simulink model "PMSM_PI"  (R2024a)
settings: Solver=FixedStepAuto  StartTime=0.0  StopTime=10  FixedStep=TsModel  RelTol=1e-3
values from neighbouring files (symbols this model uses):
  ADRC_times = 4.0    [data_PMSM_PI.sldd]
  B = 0.0    [data_PMSM_PI.sldd]
  b0 = 2000.0    [data_PMSM_PI.sldd]
  CCR_Counter = 4199.0    [data_PMSM_PI.sldd]
  CUR_I = 105.0    [data_PMSM_PI.sldd]
  CUR_P = 0.255    [data_PMSM_PI.sldd]
  current_bandwidth = 1500.0    [data_PMSM_PI.sldd]
  currunt_omega_c = 350.0    [data_PMSM_PI.sldd]
  flux = 0.00419    [data_PMSM_PI.sldd]
  Idq_limit = 20.0    [data_PMSM_PI.sldd]
  J = 5.8E-5    [data_PMSM_PI.sldd]
  Ld = 0.00017    [data_PMSM_PI.sldd]
  Lq = 0.00017    [data_PMSM_PI.sldd]
  Ls = 0.00017    [data_PMSM_PI.sldd]
  omega_c = 330.0    [data_PMSM_PI.sldd]
  omega_c_LQR = 35.0    [data_PMSM_PI.sldd]
  PMSM_CCR_Counter = 4199.0    [data_PMSM_PI.sldd]
  Pn = 5.0    [data_PMSM_PI.sldd]
  Rs = 0.07    [data_PMSM_PI.sldd]
  speed_bandwidth = 200.0    [data_PMSM_PI.sldd]
  speed_bandwidth_LQR = 60.0    [data_PMSM_PI.sldd]
  SPEED_I = 18.457    [data_PMSM_PI.sldd]
  SPEED_P = 0.18457    [data_PMSM_PI.sldd]
  Ts = 0.0001    [data_PMSM_PI.sldd]
  TsModel = 2.5E-5    [data_PMSM_PI.sldd]
  two_b0 = 2649534.0    [data_PMSM_PI.sldd]
  two_omega_c = 85.0    [data_PMSM_PI.sldd]
undefined symbols (not defined in the file or in its folder): DiscIntNeverNeededParam, sigbuilder_block
libraries: slpidlib x4, simulink x1, mcbplantlib x1, autolibpmsmexterior x1
(part 1 of 2)
settings Model: DataDictionary=data_PMSM_PI.sldd  Creator=DaLiu  LastModifiedBy=ZJH
settings OptimizationCC: DefaultParameterBehavior=Inlined  GainParamInheritBuiltInType=on  UseFloatMulNetSlope=on  UseSpecifiedMinMax=on  InlineInvariantSignals=on  EnhancedBackFolding=on  PassReuseOutputArgsAs=Individual arguments  ZeroExternalMemoryAtStartup=off  NoFixptDivByZeroProtection=on  EfficientFloat2IntCast=on  OptimizeBlockOrder=speed  DifferentSizesBufferReuse=on  OptimizationCustomize=off  EfficientTunableParamExpr=on
settings DebuggingCC: ParameterOverflowMsg=none  ParameterUnderflowMsg=error  ParameterPrecisionLossMsg=none  ParameterTunabilityLossMsg=error
settings HardwareCC: ProdBitPerPointer=32  ProdBitPerSizeT=32  ProdBitPerPtrDiffT=32  ProdLargestAtomicInteger=Long  ProdLargestAtomicFloat=Double  ProdWordSize=32  ProdHWDeviceType=ARM Compatible->ARM Cortex-M
settings SFSimCC: MATLABDynamicMemAlloc=off
settings RTWCC: Description=Embedded Coder  SystemTargetFile=ert.tlc  GenCodeOnly=on  TemplateMakefile=ert_default_tmf  RTWUseSimCustomCode=on  BuildConfiguration=Faster Runs  GPUComputeCapability=3.5
settings CodeAppCC: ForceParamTrailComments=on  GenerateComments=off  IgnoreCustomStorageClasses=off  OperatorAnnotations=on  SimulinkDataObjDesc=on  SFDataObjDesc=on  InsertBlockDesc=on
settings ERTTargetCC: TargetLangStandard=C99 (ISO)  CodeReplacementLibrary=GNU C99 extensions  GenerateSampleERTMain=on  CombineSignalStateStructs=on  SupportAbsoluteTime=off  SupportNonFinite=off  SupportComplex=off  InlinedParameterPlacement=NonHierarchical  ERTCustomFileTemplate=example_file_process.tlc  IndentSize=4

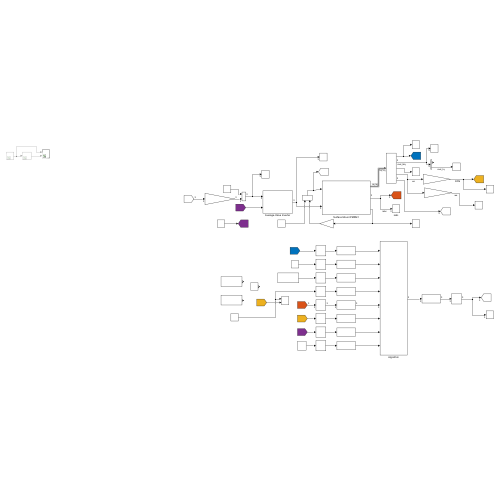
[thumbnail: Simulink's stored preview of the top-level diagram]
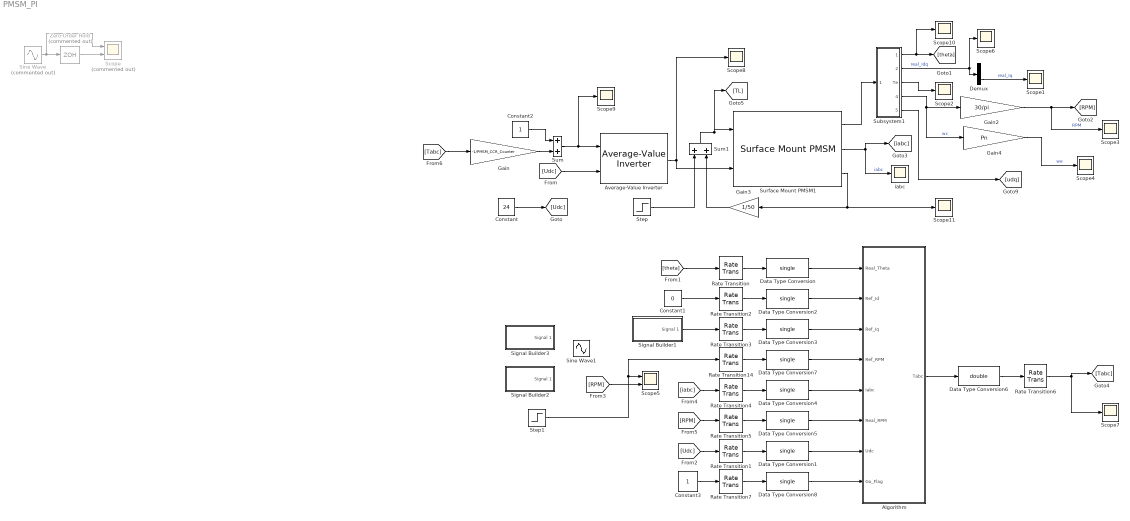
== system PMSM_PI ==
  Algorithm : Subsystem
  Average-Value Inverter : mcbplantlib/Average-Value Inverter
      settings: LibrarySourceBlock=mcblib/Electrical Systems/Inverters/Average-Value Inverter
  Constant : Constant  Value=24  SampleTime=TsModel
  Constant1 : Constant  Value=0  SampleTime=Ts
  Constant2 : Constant  SampleTime=TsModel
  Constant3 : Constant  SampleTime=Ts
  Data Type Conversion{,1..5,7..8} (8 alike) : DataTypeConversion  OutDataTypeStr=single  SaturateOnIntegerOverflow=off  RndMeth=Floor
  Data Type Conversion6 : DataTypeConversion  OutDataTypeStr=double  SaturateOnIntegerOverflow=off  RndMeth=Floor
  Demux : Demux  Outputs=2
  Gain : Gain  Gain=-1/PMSM_CCR_Counter
  Gain2 : Gain  Gain=30/pi
  Gain3 : Gain  Gain=1/50
  Gain4 : Gain  Gain=Pn
  Rate Transition{,1..5,7,14} (8 alike) : RateTransition  OutPortSampleTime=Ts
  Rate Transition6 : RateTransition  OutPortSampleTime=TsModel
  Scope : Scope  Commented=on  NumInputPorts=2
  Scope{1..4,6..11} (10 alike) : Scope
  Scope5 : Scope  NumInputPorts=2
  Signal Builder1 : Subsystem  Tag=STV Subsys  LoadFcn=sigbuilder_block('load');  StartFcn=sigbuilder_block('start');  StopFcn=sigbuilder_block('stop');  ClipboardFcn=sigbuilder_block('clipboard');  mask(Sigbuilder block){tuvar=[0:10]}
      mask help: Simulink:masks:SigbuilderBlock_MD
      mask init:
      | if ~strcmp(get_param(bdroot(gcbh),'SimulationStatus'),'stopped') tuvar = sigbuilder_block('maskInit'); end
      settings: CopyFcn=sigbuilder_block('copy');  DeleteFcn=sigbuilder_block('delete');  ModelCloseFcn=sigbuilder_block('modelClose');  PreSaveFcn=sigbuilder_block('preSave');  PauseFcn=sigbuilder_block('pause');  ContinueFcn=sigbuilder_block('continue');  NameChangeFcn=sigbuilder_block('namechange');  OpenFcn=sigbuilder_block('open',[192.6 154.8 702 251.4 ]);  CloseFcn=sigbuilder_block('close');
      mask Display: plot(0, 0, 100, 100,[2, 2, 32, 32, 2], [68, 8, 8, 68, 68],[32, 2], [38, 38], [32, 19, 2],[53, 60, 44], [32, 17, 17, 2],[16, 16, 31, 31]);txt = getActiveGroup(gcbh);text(2, 100, txt,'verticalAlignment', 'top');
  Signal Builder2 : Subsystem  Tag=STV Subsys  LoadFcn=sigbuilder_block('load');  StartFcn=sigbuilder_block('start');  StopFcn=sigbuilder_block('stop');  ClipboardFcn=sigbuilder_block('clipboard');  mask(Sigbuilder block){tuvar=[0:10]}
      mask help: Simulink:masks:SigbuilderBlock_MD
      mask init:
      | if ~strcmp(get_param(bdroot(gcbh),'SimulationStatus'),'stopped') tuvar = sigbuilder_block('maskInit'); end
      settings: CopyFcn=sigbuilder_block('copy');  DeleteFcn=sigbuilder_block('delete');  ModelCloseFcn=sigbuilder_block('modelClose');  PreSaveFcn=sigbuilder_block('preSave');  PauseFcn=sigbuilder_block('pause');  ContinueFcn=sigbuilder_block('continue');  NameChangeFcn=sigbuilder_block('namechange');  OpenFcn=sigbuilder_block('open',[205.2 81 729 231 ]);  CloseFcn=sigbuilder_block('close');
      mask Display: plot(0, 0, 100, 100,[2, 2, 32, 32, 2], [68, 8, 8, 68, 68],[32, 2], [38, 38], [32, 19, 2],[53, 60, 44], [32, 17, 17, 2],[16, 16, 31, 31]);txt = getActiveGroup(gcbh);text(2, 100, txt,'verticalAlignment', 'top');
  Signal Builder3 : Subsystem  Tag=STV Subsys  LoadFcn=sigbuilder_block('load');  StartFcn=sigbuilder_block('start');  StopFcn=sigbuilder_block('stop');  ClipboardFcn=sigbuilder_block('clipboard');  mask(Sigbuilder block){tuvar=[0:10]}
      mask help: Simulink:masks:SigbuilderBlock_MD
      mask init:
      | if ~strcmp(get_param(bdroot(gcbh),'SimulationStatus'),'stopped') tuvar = sigbuilder_block('maskInit'); end
      settings: CopyFcn=sigbuilder_block('copy');  DeleteFcn=sigbuilder_block('delete');  ModelCloseFcn=sigbuilder_block('modelClose');  PreSaveFcn=sigbuilder_block('preSave');  PauseFcn=sigbuilder_block('pause');  ContinueFcn=sigbuilder_block('continue');  NameChangeFcn=sigbuilder_block('namechange');  OpenFcn=sigbuilder_block('open',[303 127.2 729 342.6 ]);  CloseFcn=sigbuilder_block('close');
      mask Display: plot(0, 0, 100, 100,[2, 2, 32, 32, 2], [68, 8, 8, 68, 68],[32, 2], [38, 38], [32, 19, 2],[53, 60, 44], [32, 17, 17, 2],[16, 16, 31, 31]);txt = getActiveGroup(gcbh);text(2, 100, txt,'verticalAlignment', 'top');
  Sine Wave : Sin  Commented=on  SampleTime=Ts
  Sine Wave1 : Sin  Amplitude=150  SampleTime=0
  Step : Step  Time=5  After=0.1  SampleTime=Ts
  Step1 : Step  Time=0  After=100  SampleTime=Ts
  Subsystem1 : Subsystem
  Sum : Sum
  Sum1 : Sum
  Surface Mount PMSM1 : autolibpmsmexterior/Surface Mount PMSM  port_config=Torque  sim_type=Discrete  Ts=TsModel  P=Pn  Rs=Rs  Ldq_=Ls  KConstText=Permanent flux linkage constant (lambda_pm):  lambda_pm=flux  Ke=159.9771  Kt=1.323  mechanical=[J, B, 0]  idq0=[0 0]  theta_init=0  omega_init=0  KConst=flux  lambda_pm_calc=flux  RefBlkName='autolibpmsmexterior/Surface Mount PMSM'  aMode=5  Ldq="[0.0017      0.0017]"
  Zero-Order Hold : ZeroOrderHold  Commented=on
  iabc : Scope
  wires:
  Surface Mount PMSM1/1 -> Subsystem1/1(Info)
  Surface Mount PMSM1/2 -> [iabc], iabc/1  "iabc"
  Average-Value Inverter/1 -> Surface Mount PMSM1/2, Scope8/1
  Constant/1 -> [Udc]
  [Udc] -> Average-Value Inverter/2
  Subsystem1/2(I_dq) -> Demux/1, Scope6/1  "real_Idq"
  Demux/2 -> Scope1/1  "real_Iq"
  Subsystem1/3(Te) -> Scope2/1
  Subsystem1/4(Speed) -> Gain4/1, Gain2/1  "wc"
  Gain2/1 -> [RPM], Scope3/1  "RPM"
  Gain4/1 -> Scope4/1  "we"
  Subsystem1/1(Theta) -> [theta], Scope10/1
  [theta] -> Rate Transition/1
  Rate Transition/1 -> Data Type Conversion/1
  Data Type Conversion/1 -> Algorithm/1(Real_Theta)
  Data Type Conversion1/1 -> Algorithm/7(Udc)
  Rate Transition1/1 -> Data Type Conversion1/1
  [Udc] -> Rate Transition1/1
  Constant1/1 -> Rate Transition2/1
  Rate Transition2/1 -> Data Type Conversion2/1
  Data Type Conversion2/1 -> Algorithm/2(Ref_Id)
  Signal Builder1/1(Signal 1) -> Rate Transition3/1
  Data Type Conversion3/1 -> Algorithm/3(Ref_Iq)
  Rate Transition3/1 -> Data Type Conversion3/1
  Data Type Conversion7/1 -> Algorithm/4(Ref_RPM)
  Step1/1 -> Rate Transition14/1, Scope5/1
  [RPM] -> Scope5/2
  Rate Transition14/1 -> Data Type Conversion7/1
  [iabc] -> Rate Transition4/1
  Rate Transition4/1 -> Data Type Conversion4/1
  Data Type Conversion4/1 -> Algorithm/5(Iabc)
  [RPM] -> Rate Transition5/1
  Rate Transition5/1 -> Data Type Conversion5/1
  Data Type Conversion5/1 -> Algorithm/6(Real_RPM)
  Algorithm/1(Tabc) -> Data Type Conversion6/1
  Data Type Conversion6/1 -> Rate Transition6/1
  Rate Transition6/1 -> [Tabc], Scope7/1
  [Tabc] -> Gain/1
  Gain/1 -> Sum/2
  Constant2/1 -> Sum/1
  Sum/1 -> Scope9/1, Average-Value Inverter/1
  Surface Mount PMSM1/3 -> Scope11/1, Gain3/1
  Constant3/1 -> Rate Transition7/1
  Rate Transition7/1 -> Data Type Conversion8/1
  Data Type Conversion8/1 -> Algorithm/8(Go_Flag)
  Step/1 -> Sum1/1
  Gain3/1 -> Sum1/2
  Sum1/1 -> [TL], Surface Mount PMSM1/1
  Subsystem1/5(udq) -> [udq]
  Sine Wave/1 -> Scope/1, Zero-Order Hold/1
  Zero-Order Hold/1 -> Scope/2

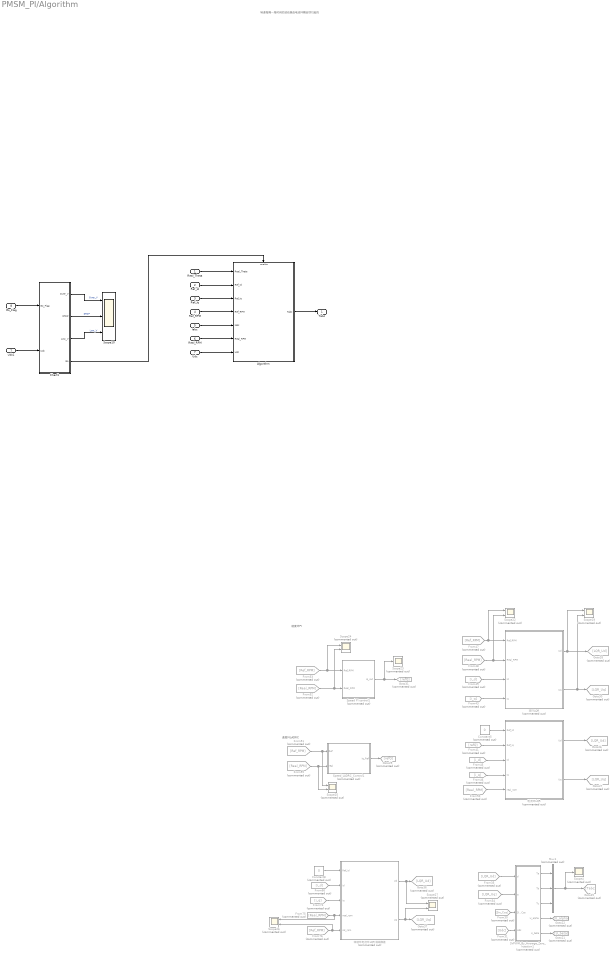
== system PMSM_PI/Algorithm ==
  note: 转速每隔一段时间的波动是由电流环耦合项引起的
  note: 速度环LADRC
  note: 速度环PI
  Real_Theta : Inport  OutDataTypeStr=single
  Ref_Id : Inport  Port=2  OutDataTypeStr=single
  Ref_Iq : Inport  Port=3  OutDataTypeStr=single
  Ref_RPM : Inport  Port=4  OutDataTypeStr=single
  Iabc : Inport  Port=5  OutDataTypeStr=single
  Real_RPM : Inport  Port=6
  Udc : Inport  Port=7  OutDataTypeStr=single
  Go_Flag : Inport  Port=8
  Algorithm : Subsystem
  Chart1 : Stateflow chart  TreatAsAtomicUnit=on
  Constant5 : Constant  Commented=on  Value=0  SampleTime=Ts
  Constant8 : Constant  Commented=on  Value=0  SampleTime=Ts
  From30 : From  Commented=on  GotoTag=Sin_Cos
  From31 : From  Commented=on  GotoTag=Udc
  From34 : From  Commented=on  GotoTag=LQR_Uq
  From35 : From  Commented=on  GotoTag=LQR_Ud
  From41 : From  Commented=on  GotoTag=refQ
  From43 : From  Commented=on  GotoTag=i_q
  From45 : From  Commented=on  GotoTag=i_d
  From46 : From  Commented=on  GotoTag=i_q
  From{47,51,53,76} (4 alike) : From  Commented=on  GotoTag=Ref_RPM
  From{48,50,52,55,75} (5 alike) : From  Commented=on  GotoTag=Real_RPM
  From49 : From  Commented=on  GotoTag=i_d
  From66 : From  Commented=on  GotoTag=i_d
  From74 : From  Commented=on  GotoTag=i_q
  Goto21 : Goto  Commented=on  GotoTag=U_beta
  Goto22 : Goto  Commented=on  GotoTag=U_alpha
  Goto25 : Goto  Commented=on  GotoTag=Tabc
  Goto26 : Goto  Commented=on  GotoTag=LQR_Ud
  Goto27 : Goto  Commented=on  GotoTag=LQR_Uq
  Goto28 : Goto  Commented=on  GotoTag=LQR_Ud
  Goto29 : Goto  Commented=on  GotoTag=refQ
  Goto30 : Goto  Commented=on  GotoTag=LQR_Uq
  Goto31 : Goto  Commented=on  GotoTag=refQ
  Goto36 : Goto  Commented=on  GotoTag=LQR_Ud
  Goto37 : Goto  Commented=on  GotoTag=LQR_Uq
  Mux1 : Mux  Commented=on  Inputs=3
  SVPWM_By_Average_Zero_Injection1 : Subsystem  Commented=on  TreatAsAtomicUnit=on
  Scope10 : Scope  NumInputPorts=3
  Scope{19,22,24..27} (6 alike) : Scope  Commented=on  NumInputPorts=2
  Scope23 : Scope  Commented=on
  Scope4 : Scope  Commented=on
  Speed PI control1 : Subsystem  Commented=on  TreatAsAtomicUnit=on
  Speed_LADRC_Control1 : Subsystem  Commented=on  TreatAsAtomicUnit=on
  Udc1 : InportShadow  Port=7  OutDataTypeStr=single
  双环LQR : Subsystem  Commented=on
  电流环LQR : Subsystem  Commented=on
  转速环电流环LQR消除静差 : Subsystem  Commented=on
  Tabc : Outport  OutDataTypeStr=single
  wires:
  Udc/1 -> Algorithm/7(Udc)
  Real_Theta/1 -> Algorithm/1(Real_Theta)
  Ref_RPM/1 -> Algorithm/4(Ref_RPM)
  Ref_Iq/1 -> Algorithm/3(Ref_Iq)
  Iabc/1 -> Algorithm/5(Iabc)
  Real_RPM/1 -> Algorithm/6(Real_RPM)
  Mux1/1 -> Goto25/1, Scope4/1
  SVPWM_By_Average_Zero_Injection1/3(Tc) -> Mux1/3
  SVPWM_By_Average_Zero_Injection1/5(U_beta) -> Goto21/1
  SVPWM_By_Average_Zero_Injection1/2(Tb) -> Mux1/2
  SVPWM_By_Average_Zero_Injection1/4(U_alpha) -> Goto22/1
  SVPWM_By_Average_Zero_Injection1/1(Ta) -> Mux1/1
  From35/1 -> SVPWM_By_Average_Zero_Injection1/1(d)
  From30/1 -> SVPWM_By_Average_Zero_Injection1/3(Sin&Cos)
  From31/1 -> SVPWM_By_Average_Zero_Injection1/4(Udc)
  From34/1 -> SVPWM_By_Average_Zero_Injection1/2(q)
  Algorithm/1(Tabc) -> Tabc/1
  From48/1 -> Scope22/2, 双环LQR/2(Real_RPM)
  From47/1 -> Scope22/1, 双环LQR/1(Ref_RPM)
  From49/1 -> 双环LQR/3(id)
  From43/1 -> 双环LQR/4(iq)
  双环LQR/2(Uq) -> Scope19/2, Goto30/1
  双环LQR/1(Ud) -> Scope19/1, Goto28/1
  电流环LQR/1(Ud) -> Goto26/1
  电流环LQR/2(Uq) -> Goto27/1
  From41/1 -> 电流环LQR/2(Ref_iq)
  Constant5/1 -> 电流环LQR/1(Ref_id)
  From45/1 -> 电流环LQR/3(id)
  From46/1 -> 电流环LQR/4(iq)
  From50/1 -> 电流环LQR/5(real_rpm)
  From52/1 -> Speed PI control1/2(Real_RPM), Scope24/2
  From53/1 -> Speed PI control1/1(Ref_RPM), Scope24/1
  From51/1 -> Speed_LADRC_Control1/1(Ref), Scope25/1
  Speed PI control1/1(Iq_out) -> Goto31/1, Scope23/1
  From55/1 -> Scope25/2, Speed_LADRC_Control1/2(real)
  Speed_LADRC_Control1/1(Iq_Ref) -> Goto29/1
  From76/1 -> Scope26/2, 转速环电流环LQR消除静差/5(rel_rpm)
  From75/1 -> Scope26/1, 转速环电流环LQR消除静差/4(real_rpm)
  From74/1 -> 转速环电流环LQR消除静差/3(iq)
  From66/1 -> 转速环电流环LQR消除静差/2(id)
  Constant8/1 -> 转速环电流环LQR消除静差/1(Ref_id)
  转速环电流环LQR消除静差/2(Uq) -> Scope27/2, Goto37/1
  转速环电流环LQR消除静差/1(Ud) -> Scope27/1, Goto36/1
  Go_Flag/1 -> Chart1/1(Go_Flag)
  Chart1/3(Low_V) -> Scope10/3  "Low_V"
  Chart1/2(STOP) -> Scope10/2  "STOP"
  Chart1/1(Over_V) -> Scope10/1  "Over_V"
  Udc1/1 -> Chart1/2(Udc)
  Chart1/4(Go) -> Algorithm/Enable
  Ref_Id/1 -> Algorithm/2(Ref_Id)

== system PMSM_PI/Signal Builder1 ==
  Demux : Demux  Tag=STV Demux  Outputs=1
      settings: DisplayOption=none
  FromWs : FromWorkspace  Tag=STV FromWs  VariableName=tuvar
      SigBuilderData=|
      | common.afterFinalStr = 'Extrapolate'
      | common.sampleTime = 0
      | dataSet.timeRange = [0 10]
      | dataSet.name = 'Group 1'
      | sbobj.Groups.Name = 'Group 1'
      | sbobj.Groups.Signals.Name = 'Signal 1'
      | sbobj.Groups.Signals.XData = [0 1.9 1.9 3.56 3.56 10]
      | sbobj.Groups.Signals.YData = [5 5 7.2 7.2 8 8]
  Signal 1 : Outport  Tag=STV Outport
  wires:
  Demux/1 -> Signal 1/1
  FromWs/1 -> Demux/1

== system PMSM_PI/Signal Builder2 ==
  Demux : Demux  Tag=STV Demux  Outputs=1
      settings: DisplayOption=none
  FromWs : FromWorkspace  Tag=STV FromWs  VariableName=tuvar
      SigBuilderData=|
      | common.afterFinalStr = 'Extrapolate'
      | common.sampleTime = 0
      | dataSet.timeRange = [0 10]
      | dataSet.name = 'Group 1'
      | sbobj.Groups.Name = 'Group 1'
      | sbobj.Groups.Signals.Name = 'Signal 1'
      | sbobj.Groups.Signals.XData = [0 3 6.02 10]
      | sbobj.Groups.Signals.YData = [150 150 250 200]
  Signal 1 : Outport  Tag=STV Outport
  wires:
  Demux/1 -> Signal 1/1
  FromWs/1 -> Demux/1

== system PMSM_PI/Signal Builder3 ==
  Demux : Demux  Tag=STV Demux  Outputs=1
      settings: DisplayOption=none
  FromWs : FromWorkspace  Tag=STV FromWs  VariableName=tuvar
      SigBuilderData=|
      | common.afterFinalStr = 'Extrapolate'
      | common.sampleTime = 0
      | dataSet.timeRange = [0 10]
      | dataSet.name = 'Group 1'
      | sbobj.Groups.Name = 'Group 1'
      | sbobj.Groups.Signals.Name = 'Signal 1'
      | sbobj.Groups.Signals.XData = [0 3 3 6.02 6.02 10]
      | sbobj.Groups.Signals.YData = [150 150 250 250 200 200]
  Signal 1 : Outport  Tag=STV Outport
  wires:
  FromWs/1 -> Demux/1
  Demux/1 -> Signal 1/1

== system PMSM_PI/Subsystem1 ==
  Info : Inport
  Bus Selector2 : BusSelector  OutputSignals=IdSync,IqSync,MtrPos,MtrTrq,MtrSpd,VdSync,VqSync
  Constant4 : Constant  Value=2*pi  SampleTime=-1
  Gain2 : Gain  Gain=Pn
  Mod1 : Math  Operator=mod
  Mux : Mux  Inputs=2
  Mux1 : Mux  Inputs=2
  Scope : Scope
  Theta : Outport
  I_dq : Outport  Port=2
  Te : Outport  Port=3
  Speed : Outport  Port=4
  udq : Outport  Port=5
  wires:
  Bus Selector2/2 -> Mux/2  "<IqSync>"
  Gain2/1 -> Mod1/1
  Mod1/1 -> Theta/1
  Bus Selector2/1 -> Mux/1  "<IdSync>"
  Constant4/1 -> Mod1/2
  Info/1 -> Bus Selector2/1
  Bus Selector2/3 -> Gain2/1  "<MtrPos>"
  Mux/1 -> I_dq/1
  Bus Selector2/4 -> Te/1  "<MtrTrq>"
  Bus Selector2/5 -> Scope/1, Speed/1  "<MtrSpd>"
  Bus Selector2/6 -> Mux1/1  "<VdSync>"
  Bus Selector2/7 -> Mux1/2  "<VqSync>"
  Mux1/1 -> udq/1

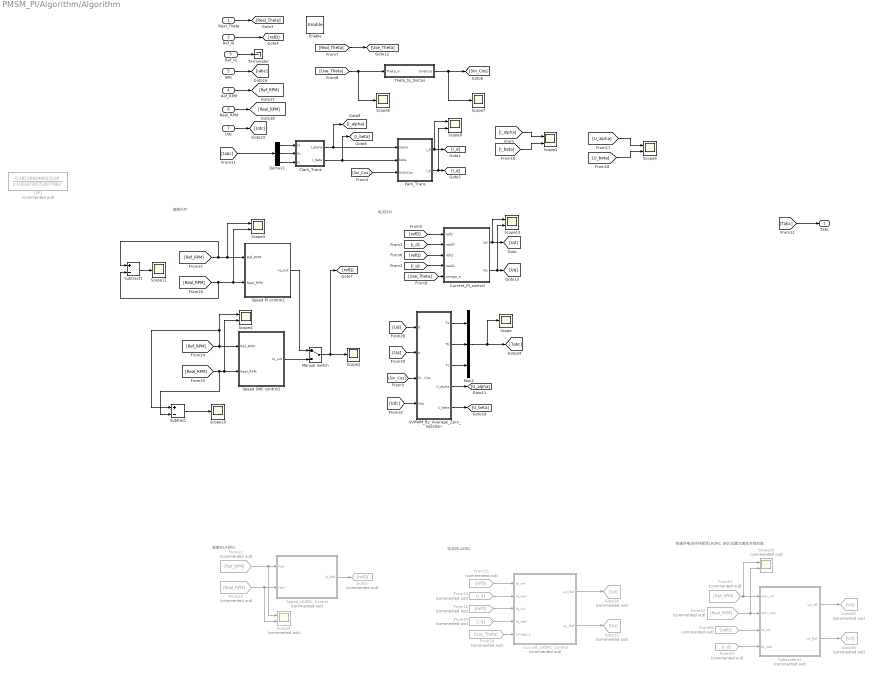
== system PMSM_PI/Algorithm/Algorithm ==
  note: 电流环PI
  note: 速度环PI
  note: 转速环电流环并联双LADRC
      | 该b0设置为真实方程的值
  note: 电流环LADRC
  note: 速度环LADRC
  Real_Theta : Inport  OutDataTypeStr=single
  Ref_Id : Inport  Port=2  OutDataTypeStr=single
  Ref_Iq : Inport  Port=3  OutDataTypeStr=single
  Ref_RPM : Inport  Port=4  OutDataTypeStr=single
  Iabc : Inport  Port=5  OutDataTypeStr=single
  Real_RPM : Inport  Port=6
  Udc : Inport  Port=7  OutDataTypeStr=single
  Enable : EnablePort
  Clark_Trans : Subsystem  TreatAsAtomicUnit=on
      settings: RTWFcnNameOpts=Use subsystem name
  Current_PI_control : Subsystem  TreatAsAtomicUnit=on
      settings: RTWFcnNameOpts=Use subsystem name
  Currunt_LADRC_Control : Subsystem  Commented=on
  Demux1 : Demux  Outputs=3
  From13 : From  Commented=on  GotoTag=i_d
  From14 : From  Commented=on  GotoTag=i_q
  From15 : From  Commented=on  GotoTag=refD
  From16 : From  Commented=on  GotoTag=refQ
  From19 : From  Commented=on  GotoTag=Use_Theta
  From22 : From  Commented=on  GotoTag=Ref_RPM
  From23 : From  Commented=on  GotoTag=Real_RPM
  From37 : From  Commented=on  GotoTag=Real_RPM
  From54 : From  Commented=on  GotoTag=Ref_RPM
  From56 : From  Commented=on  GotoTag=refD
  From57 : From  Commented=on  GotoTag=i_d
  Goto14 : Goto  Commented=on  GotoTag=Ud
  Goto15 : Goto  Commented=on  GotoTag=Uq
  Goto38 : Goto  Commented=on  GotoTag=Ud
  Goto39 : Goto  Commented=on  GotoTag=Uq
  Goto5 : Goto  Commented=on  GotoTag=refQ
  LPF1 : DiscreteTransferFcn  Commented=on  Numerator=[0.181269246922018]  Denominator=[1 -0.818730753077982]
  Manual Switch : ManualSwitch
  Mux2 : Mux  Inputs=3
  Park_Trans : Subsystem  TreatAsAtomicUnit=on
      settings: RTWFcnNameOpts=Use subsystem name
  SVPWM_By_Average_Zero_Injection : Subsystem  TreatAsAtomicUnit=on
  Scope{,2,6..7,10..11} (6 alike) : Scope
  Scope{1,3..4,8..9,13} (6 alike) : Scope  NumInputPorts=2
  Scope29 : Scope  Commented=on  NumInputPorts=2
  Scope5 : Scope  Commented=on  NumInputPorts=2
  Speed PI control2 : Subsystem  TreatAsAtomicUnit=on
  Speed SMC control1 : Subsystem  TreatAsAtomicUnit=on
  Speed_LADRC_Control : Subsystem  Commented=on  TreatAsAtomicUnit=on
  Subsystem1 : Subsystem  Commented=on
  Subtract : Sum  Inputs=+-
  Subtract1 : Sum  Inputs=+-
  Terminator : Terminator
  Theta_to_SinCos : Subsystem  TreatAsAtomicUnit=on
  Tabc : Outport
  wires:
  [i_d] -> Current_PI_control/2(realD)
  [refQ] -> Current_PI_control/3(refQ)
  [Udc] -> SVPWM_By_Average_Zero_Injection/4(Udc)
  SVPWM_By_Average_Zero_Injection/3(Tc) -> Mux2/3
  Current_PI_control/1(Ud) -> Scope13/1, [Ud]
  [Uq] -> SVPWM_By_Average_Zero_Injection/2(q)
  [refD] -> Current_PI_control/1(refD)
  [Sin_Cos] -> SVPWM_By_Average_Zero_Injection/3(Sin&Cos)
  Mux2/1 -> [Tabc], Scope/1
  SVPWM_By_Average_Zero_Injection/4(U_alpha) -> [U_alpha]
  Current_PI_control/2(Uq) -> Scope13/2, [Uq]
  [Ud] -> SVPWM_By_Average_Zero_Injection/1(d)
  [Ref_RPM] -> Subtract1/1, Scope3/1, Speed PI control2/1(Ref_RPM)
  SVPWM_By_Average_Zero_Injection/1(Ta) -> Mux2/1
  [i_q] -> Current_PI_control/4(realQ)
  [Real_RPM] -> Speed PI control2/2(Real_RPM), Scope3/2, Subtract1/2
  SVPWM_By_Average_Zero_Injection/5(U_beta) -> [U_beta]
  SVPWM_By_Average_Zero_Injection/2(Tb) -> Mux2/2
  [Use_Theta] -> Current_PI_control/5(omega_e)
  [Sin_Cos] -> Park_Trans/3(Sin&Cos)
  Clark_Trans/1(I_alpha) -> [I_alpha], Park_Trans/1(alpha)
  [I_alpha] -> Scope1/1
  Park_Trans/1(i_d) -> Scope8/1, [i_d]
  Clark_Trans/2(I_beta) -> Park_Trans/2(beta), [I_beta]
  Demux1/1 -> Clark_Trans/1(Ia)
  [Use_Theta] -> Scope6/1, Theta_to_SinCos/1(Theta_in)
  [Real_Theta] -> [Use_Theta]
  Theta_to_SinCos/1(Sin&Cos) -> Scope7/1, [Sin_Cos]
  [U_alpha] -> Scope9/1
  Park_Trans/2(i_q) -> Scope8/2, [i_q]
  Demux1/3 -> Clark_Trans/3(Ic)
  [U_beta] -> Scope9/2
  Demux1/2 -> Clark_Trans/2(Ib)
  [I_beta] -> Scope1/2
  Ref_Id/1 -> [refD]
  Real_Theta/1 -> [Real_Theta]
  Ref_Iq/1 -> Terminator/1
  Iabc/1 -> [Iabc]
  Real_RPM/1 -> [Real_RPM]
  Ref_RPM/1 -> [Ref_RPM]
  Udc/1 -> [Udc]
  [Tabc] -> Tabc/1
  From16/1 -> Currunt_LADRC_Control/3(Iq_ref)
  From14/1 -> Currunt_LADRC_Control/4(Iq_real)
  Speed_LADRC_Control/1(Iq_Ref) -> Goto5/1
  From54/1 -> Scope29/1, Subsystem1/1(rpm_ref)
  Subsystem1/1(uq_ref) -> Goto39/1
  From23/1 -> Speed_LADRC_Control/2(real), Scope5/2
  From57/1 -> Subsystem1/4(Id_real)
  From37/1 -> Scope29/2, Subsystem1/2(rpm_real)
  From13/1 -> Currunt_LADRC_Control/2(Id_real)
  From22/1 -> Scope5/1, Speed_LADRC_Control/1(Ref)
  From19/1 -> Currunt_LADRC_Control/5(omega_e)
  Subsystem1/2(ud_Ref) -> Goto38/1
  Currunt_LADRC_Control/2(uq_Ref) -> Goto15/1
  From15/1 -> Currunt_LADRC_Control/1(Id_ref)
  Currunt_LADRC_Control/1(ud_Ref) -> Goto14/1
  From56/1 -> Subsystem1/3(Id_ref)
  [Iabc] -> Demux1/1
  Speed PI control2/1(Iq_out) -> Manual Switch/1
  Manual Switch/1 -> [refQ], Scope2/1
  Speed SMC control1/1(Iq_out) -> Manual Switch/2
  [Real_RPM] -> Subtract/2, Scope4/2, Speed SMC control1/2(Real_RPM)
  [Ref_RPM] -> Scope4/1, Subtract/1, Speed SMC control1/1(Ref_RPM)
  Subtract/1 -> Scope10/1
  Subtract1/1 -> Scope11/1

== system PMSM_PI/Algorithm/Chart1/Low_judge ==
  Input : Inport  OutDataTypeStr=single  PortDimensions=1
  f : TriggerPort  TriggerType=function-call  VariantControl=(inherit)
      settings: CopyFcn=Stateflow.SLINSF.SimulinkMan.removeBlockPreDeleteFcn  PreDeleteFcn=Stateflow.SLINSF.SimulinkMan.unsafePredeleteFcn
  Data Type Conversion : DataTypeConversion  OutDataTypeStr=boolean  SaturateOnIntegerOverflow=off  RndMeth=Floor
  Data Type Conversion1 : DataTypeConversion  OutDataTypeStr=single  SaturateOnIntegerOverflow=off  RndMeth=Floor
  NOR : Logic  Operator=NOT  IconShape=distinctive  OutDataTypeStr=boolean
  Relay : Relay  OnSwitchValue=20  OffSwitchValue=18  OutDataTypeStr=single
  Out : Outport  OutDataTypeStr=single
  wires:
  Input/1 -> Relay/1
  Relay/1 -> Data Type Conversion/1
  NOR/1 -> Data Type Conversion1/1
  Data Type Conversion/1 -> NOR/1
  Data Type Conversion1/1 -> Out/1

== system PMSM_PI/Algorithm/Chart1/Over_judge ==
  Input : Inport  OutDataTypeStr=single  PortDimensions=1
  f : TriggerPort  TriggerType=function-call  VariantControl=(inherit)
      settings: CopyFcn=Stateflow.SLINSF.SimulinkMan.removeBlockPreDeleteFcn  PreDeleteFcn=Stateflow.SLINSF.SimulinkMan.unsafePredeleteFcn
  Relay : Relay  OnSwitchValue=28  OffSwitchValue=25  OutDataTypeStr=single
  Out : Outport  OutDataTypeStr=single
  wires:
  Input/1 -> Relay/1
  Relay/1 -> Out/1

== system PMSM_PI/Algorithm/SVPWM_By_Average_Zero_Injection1 ==
  d : Inport  OutDataTypeStr=single
  q : Inport  Port=2  OutDataTypeStr=single
  Sin&Cos : Inport  Port=3  OutDataTypeStr=single
  Udc : Inport  Port=4  OutDataTypeStr=single
  Anti_Park_Trans : Subsystem
  Gain : Gain  Gain=CCR_Counter  OutDataTypeStr=single
  Gain1 : Gain  Gain=CCR_Counter  OutDataTypeStr=single
  Gain2 : Gain  Gain=CCR_Counter  OutDataTypeStr=single
  SVPWM : Subsystem
  Scope : Scope  NumInputPorts=3
  Ta : Outport  OutDataTypeStr=single
  Tb : Outport  Port=2  OutDataTypeStr=single
  Tc : Outport  Port=3  OutDataTypeStr=single
  U_alpha : Outport  Port=4  OutDataTypeStr=single
  U_beta : Outport  Port=5  OutDataTypeStr=single
  wires:
  Anti_Park_Trans/1(alpha) -> U_alpha/1, SVPWM/1(alpha)
  q/1 -> Anti_Park_Trans/2(q)
  SVPWM/1(Ta) -> Scope/1, Gain/1
  Anti_Park_Trans/2(beta) -> U_beta/1, SVPWM/2(beta)
  d/1 -> Anti_Park_Trans/1(d)
  Sin&Cos/1 -> Anti_Park_Trans/3(Sin&Cos)
  SVPWM/2(Tb) -> Scope/2, Gain1/1
  SVPWM/3(Tc) -> Gain2/1, Scope/3
  Udc/1 -> SVPWM/3(Udc)
  Gain/1 -> Ta/1
  Gain1/1 -> Tb/1
  Gain2/1 -> Tc/1

== system PMSM_PI/Algorithm/Speed PI control1 ==
  Ref_RPM : Inport  OutDataTypeStr=single
  Real_RPM : Inport  Port=2  OutDataTypeStr=single
  Add : Sum  Inputs=+-  OutDataTypeStr=single
  Constant1 : Constant  Value=speed_bandwidth_LQR  OutDataTypeStr=single  SampleTime=Ts
  Constant2 : Constant  Value=speed_bandwidth_LQR  OutDataTypeStr=single  SampleTime=Ts
  Constant3 : Constant  Value=B  OutDataTypeStr=single  SampleTime=Ts
  Constant4 : Constant  Value=1.5*Pn*flux  OutDataTypeStr=single  SampleTime=Ts
  Divide : Product  Inputs=*/  OutDataTypeStr=single
  Gain : Gain  Gain=J/(1.5*Pn*flux)  OutDataTypeStr=single
  Gain1 : Gain  Gain=J/(1.5*Pn*flux)  OutDataTypeStr=single
  Gain2 : Gain  Gain=J  OutDataTypeStr=single
  PID Controller : slpidlib/PID Controller  Controller=PI  Form=Parallel  TimeDomain=Discrete-time  UseExternalTs=off  SampleTime=Ts  IntegratorMethod=Forward Euler  FilterMethod=Forward Euler  ControllerParametersSource=external  P=1  I=1  UseKiTs=off  D=0  UseExternalDerivativeSource=off  N=100  UseFilter=on  TunerSelectOption=Transfer Function Based (PID Tuner App)  ZeroCross=off  InitialConditionSource=internal  InitialConditionForIntegrator=1  InitialConditionForFilter=0  DifferentiatorICPrevScaledInput=0  ExternalReset=none  TrackingMode=off  Kt=1  LimitOutput=off  SatLimitsSource=internal  UpperSaturationLimit=200  LowerSaturationLimit=-200  LinearizeAsGain=on  AntiWindupMode=none  Kb=1  LimitIntegrator=off  UpperIntegratorSaturationLimit=inf  LowerIntegratorSaturationLimit=-inf  POutMin=[]  POutMax=[]  IOutMin=[]  IOutMax=[]  DOutMin=[]  DOutMax=[]  NOutMin=[]  NOutMax=[]  SumOutMin=[]  SumOutMax=[]  SaturationOutMin=[]  SaturationOutMax=[]  PParamMin=[]  PParamMax=[]  IParamMin=[]  IParamMax=[]  DParamMin=[]  DParamMax=[]  NParamMin=[]  NParamMax=[]  KbParamMin=[]  KbParamMax=[]  KtParamMin=[]  KtParamMax=[]  KbOutMin=[]  KbOutMax=[]  KtOutMin=[]  KtOutMax=[]  IntegratorOutMin=[]  IntegratorOutMax=[]  FilterOutMin=[]  FilterOutMax=[]  SumI1OutMin=[]  SumI1OutMax=[]  SumI2OutMin=[]  SumI2OutMax=[]  SumI3OutMin=[]  SumI3OutMax=[]  SumI4OutMin=[]  SumI4OutMax=[]  SumDOutMin=[]  SumDOutMax=[]  DifferentiatorOutMin=[]  DifferentiatorOutMax=[]  FilterDiffOutCoefMin=[]  FilterDiffOutCoefMax=[]  ReciprocalOutMin=[]  ReciprocalOutMax=[]  SumDenOutMin=[]  SumDenOutMax=[]  SumNumOutMin=[]  SumNumOutMax=[]  DivideOutMin=[]  DivideOutMax=[]  UdiffTsProdOutMin=[]  UdiffTsProdOutMax=[]  NTsProdOutMin=[]  NTsProdOutMax=[]  UintegralTsProdOutMin=[]  UintegralTsProdOutMax=[]  UngainTsProdOutMin=[]  UngainTsProdOutMax=[]  ClampingZeroOutDataTypeStr=Inherit: Inherit via back propagation  ClampingZeroOutMin=[]  ClampingZeroOutMax=[]  FilterDenConstantOutDataTypeStr=Inherit: Inherit via back propagation  FilterDenConstantOutMin=[]  FilterDenConstantOutMax=[]  PCopyOutDataTypeStr=Inherit: Inherit via back propagation  PCopyOutMin=[]  PCopyOutMax=[]  NCopyOutDataTypeStr=Inherit: Inherit via back propagation  NCopyOutMin=[]  NCopyOutMax=[]  IntegratorContinuousStateAttributes=''  IntegratorStateMustResolveToSignalObject=off  IntegratorRTWStateStorageClass=Auto  FilterContinuousStateAttributes=''  FilterStateMustResolveToSignalObject=off  FilterRTWStateStorageClass=Auto  ParallelPVariant=ExternalParameters  IdealPVariant=Disabled  IVariant=ExternalParameters  DVariant=Disabled  IntegratorVariant=Discrete  SatVariant=Disabled  AWVariant=Passthrough  PCopyVariant=Disabled  TRVariant=Disabled  FdbkBlocksVariant=Forward  IdealPFdbkVariant=Disabled  SatFdbkVariant=Disabled  DerivativeFilterVariant=Disabled  NVariant=Disabled  NCopyVariant=Disabled_SignalSpec  FilterICVariant=Disabled  IntegratorICVariant=InternalICs  ExternalResetVariant=Disabled  TRSumVariant=Passthrough  SumFdbkVariant=Disabled  SumVariant=Sum_PI  TsampFilterVariant=InternalTs  TsampNgainVariant=Passthrough  TsampIntegralVariant=Disabled_SignalSpec  ExternalSaturationOutDataTypeStr=Inherit: Same as second input  DerivativeSourceVariant=Disabled
  Product : Product  OutDataTypeStr=single
  Product1 : Product  OutDataTypeStr=single
  Saturation2 : Saturate  UpperLimit=Idq_limit  LowerLimit=-Idq_limit  OutDataTypeStr=single
  Step : Step  Time=8  After=0  SampleTime=Ts
  Sum : Sum  Inputs=|++
  Sum1 : Sum  Inputs=|+-  OutDataTypeStr=single
  Sum2 : Sum  Inputs=|+-  OutDataTypeStr=single
  Iq_out : Outport  OutDataTypeStr=single
  wires:
  Step/1 -> Sum/2
  Sum/1 -> Saturation2/1
  Saturation2/1 -> Iq_out/1
  Sum2/1 -> Sum/1
  Product1/1 -> Sum2/2
  Divide/1 -> Product1/1
  Constant4/1 -> Divide/2
  Add/1 -> Divide/1
  Constant3/1 -> Add/2
  Gain2/1 -> Add/1
  Product/1 -> Gain1/1
  Gain1/1 -> PID Controller/3
  Constant2/1 -> Product/1, Product/2, Gain2/1
  PID Controller/1 -> Sum2/1
  Real_RPM/1 -> Product1/2, Sum1/2
  Sum1/1 -> PID Controller/1
  Ref_RPM/1 -> Sum1/1
  Gain/1 -> PID Controller/2
  Constant1/1 -> Gain/1

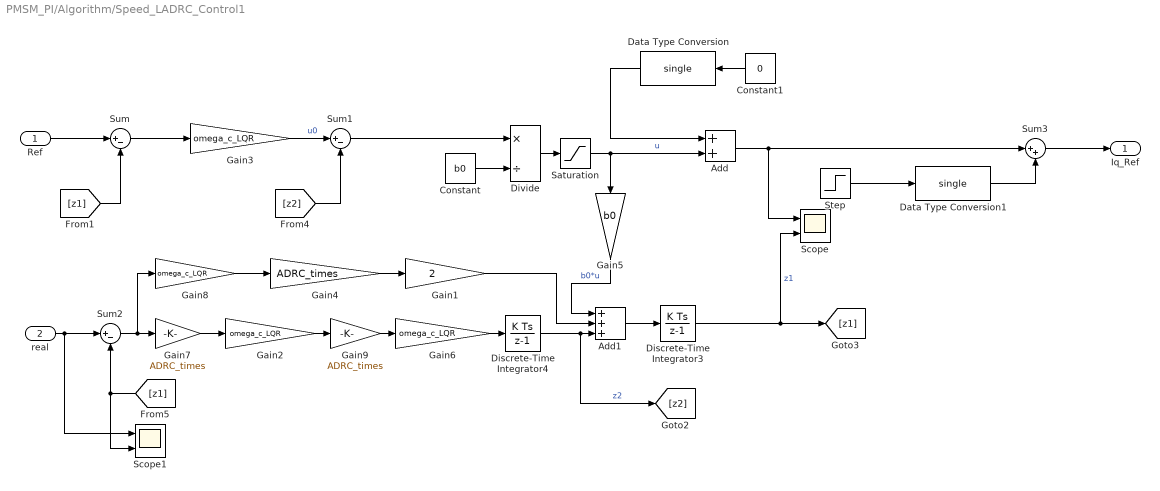
== system PMSM_PI/Algorithm/Speed_LADRC_Control1 ==
  Ref : Inport  OutDataTypeStr=single
  real : Inport  Port=2  OutDataTypeStr=single
  Add : Sum  OutDataTypeStr=single
  Add1 : Sum  Inputs=+++  OutDataTypeStr=single
  Constant : Constant  Value=b0  OutDataTypeStr=single
  Constant1 : Constant  Value=0  SampleTime=-1
  Data Type Conversion : DataTypeConversion  OutDataTypeStr=single  SaturateOnIntegerOverflow=off  RndMeth=Floor
  Data Type Conversion1 : DataTypeConversion  OutDataTypeStr=single  SaturateOnIntegerOverflow=off  RndMeth=Floor
  Discrete-Time Integrator3 : DiscreteIntegrator  SampleTime=-1  OutDataTypeStr=single  ICPrevOutput=DiscIntNeverNeededParam  ICPrevScaledInput=DiscIntNeverNeededParam
  Discrete-Time Integrator4 : DiscreteIntegrator  SampleTime=-1  OutDataTypeStr=single  ICPrevOutput=DiscIntNeverNeededParam  ICPrevScaledInput=DiscIntNeverNeededParam
  Divide : Product  Inputs=*/  OutDataTypeStr=single
  Gain1 : Gain  Gain=2  OutDataTypeStr=single
  Gain{2..3,6,8} (4 alike) : Gain  Gain=omega_c_LQR  OutDataTypeStr=single
  Gain4 : Gain  Gain=ADRC_times  OutDataTypeStr=single
  Gain5 : Gain  Gain=b0  OutDataTypeStr=single
  Gain7 : Gain  Gain=ADRC_times  OutDataTypeStr=single
  Gain9 : Gain  Gain=ADRC_times  OutDataTypeStr=single
  Saturation : Saturate  UpperLimit=Idq_limit  LowerLimit=-Idq_limit  OutDataTypeStr=single
  Scope : Scope  NumInputPorts=2
  Scope1 : Scope  NumInputPorts=2
  Step : Step  Time=8  After=0  SampleTime=Ts
  Sum : Sum  Inputs=|+-  OutDataTypeStr=single
  Sum1 : Sum  Inputs=|+-  OutDataTypeStr=single
  Sum2 : Sum  Inputs=|+-  OutDataTypeStr=single
  Sum3 : Sum  Inputs=|++
  Iq_Ref : Outport  OutDataTypeStr=single
  wires:
  Data Type Conversion1/1 -> Sum3/2
  Step/1 -> Data Type Conversion1/1
  Sum3/1 -> Iq_Ref/1
  Constant1/1 -> Data Type Conversion/1
  Gain9/1 -> Gain6/1
  Gain8/1 -> Gain4/1
  Gain7/1 -> Gain2/1
  Gain6/1 -> Discrete-Time Integrator4/1
  Gain4/1 -> Gain1/1
  Saturation/1 -> Gain5/1, Add/2  "u"
  Data Type Conversion/1 -> Add/1
  Add/1 -> Sum3/1, Scope/1
  Sum1/1 -> Divide/1
  Gain3/1 -> Sum1/1  "u0"
  Divide/1 -> Saturation/1
  Constant/1 -> Divide/2
  [z2] -> Sum1/2
  Sum/1 -> Gain3/1
  [z1] -> Sum/2
  [z1] -> Sum2/2, Scope1/2
  real/1 -> Sum2/1, Scope1/1
  Sum2/1 -> Gain8/1, Gain7/1
  Add1/1 -> Discrete-Time Integrator3/1
  Discrete-Time Integrator3/1 -> [z1], Scope/2  "z1"
  Gain1/1 -> Add1/2
  Gain2/1 -> Gain9/1
  Gain5/1 -> Add1/1  "b0*u"
  Discrete-Time Integrator4/1 -> [z2], Add1/3  "z2"
  Ref/1 -> Sum/1

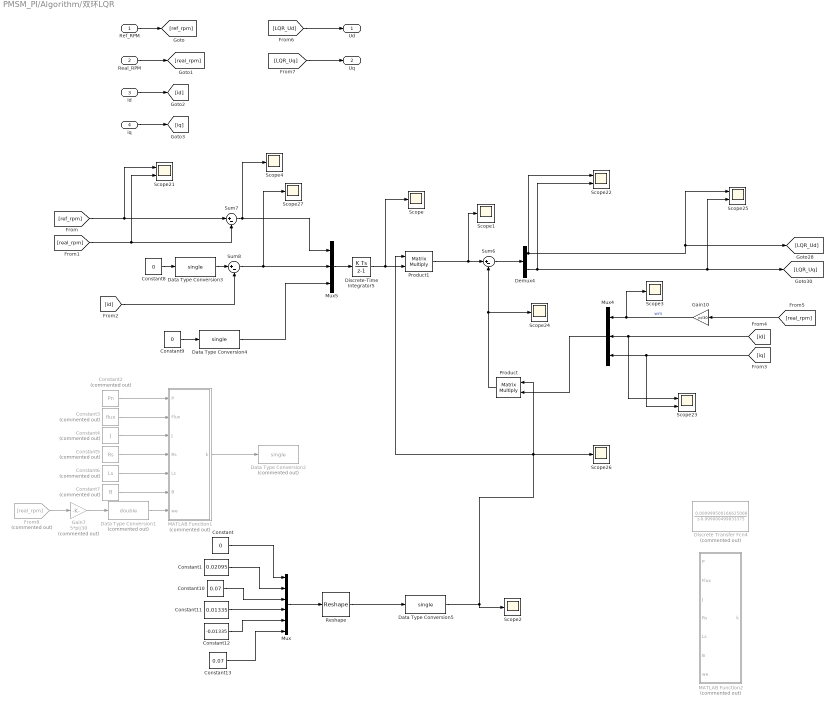
== system PMSM_PI/Algorithm/双环LQR ==
  Ref_RPM : Inport
  Real_RPM : Inport  Port=2
  id : Inport  Port=3
  iq : Inport  Port=4
  Constant : Constant  Value=0  SampleTime=Ts
  Constant1 : Constant  Value=0.02095  SampleTime=Ts
  Constant10 : Constant  Value=0.07  SampleTime=Ts
  Constant11 : Constant  Value=0.01335  SampleTime=Ts
  Constant12 : Constant  Value=-0.01335  SampleTime=Ts
  Constant13 : Constant  Value=0.07  SampleTime=Ts
  Constant2 : Constant  Commented=on  Value=Pn  SampleTime=Ts
  Constant3 : Constant  Commented=on  Value=flux  SampleTime=Ts
  Constant4 : Constant  Commented=on  Value=J  SampleTime=Ts
  Constant5 : Constant  Commented=on  Value=Rs  SampleTime=Ts
  Constant6 : Constant  Commented=on  Value=Ls  SampleTime=Ts
  Constant7 : Constant  Commented=on  Value=B  SampleTime=Ts
  Constant8 : Constant  Value=0  SampleTime=Ts
  Constant9 : Constant  Value=0  SampleTime=Ts
  Data Type Conversion1 : DataTypeConversion  Commented=on  OutDataTypeStr=double  SaturateOnIntegerOverflow=off  RndMeth=Floor
  Data Type Conversion2 : DataTypeConversion  Commented=on  OutDataTypeStr=single  SaturateOnIntegerOverflow=off  RndMeth=Floor
  Data Type Conversion3 : DataTypeConversion  OutDataTypeStr=single  SaturateOnIntegerOverflow=off  RndMeth=Floor
  Data Type Conversion4 : DataTypeConversion  OutDataTypeStr=single  SaturateOnIntegerOverflow=off  RndMeth=Floor
  Data Type Conversion5 : DataTypeConversion  OutDataTypeStr=single  SaturateOnIntegerOverflow=off  RndMeth=Floor
  Demux4 : Demux  Outputs=2
  Discrete Transfer Fcn4 : DiscreteTransferFcn  Commented=on  Numerator=[0.000999500166625008]  Denominator=[1 -0.999000499833375]
  Discrete-Time Integrator5 : DiscreteIntegrator  gainval=90  SampleTime=-1  ICPrevOutput=DiscIntNeverNeededParam  ICPrevScaledInput=DiscIntNeverNeededParam
  From8 : From  Commented=on  GotoTag=real_rpm
  Gain10 : Gain  Gain=pi/30
  Gain7 : Gain  Commented=on  Gain=5*pi/30
  MATLAB Function1 : MATLAB Function  Commented=on  TreatAsAtomicUnit=on
  MATLAB Function2 : MATLAB Function  Commented=on  TreatAsAtomicUnit=on
  Mux : Mux  Inputs=6
  Mux4 : Mux  Inputs=3
  Mux5 : Mux  Inputs=3
  Product : Product  Multiplication=Matrix(*)
  Product1 : Product  Multiplication=Matrix(*)
  Reshape : Reshape  OutputDimensionality=Customize  OutputDimensions=[2,3]
  Scope{,1..4,24,26..27} (8 alike) : Scope
  Scope{21..23,25} (4 alike) : Scope  NumInputPorts=2
  Sum6 : Sum  Inputs=|+-
  Sum7 : Sum  Inputs=|+-
  Sum8 : Sum  Inputs=|+-
  Ud : Outport
  Uq : Outport  Port=2
  wires:
  Constant5/1 -> MATLAB Function1/4(Rs)
  Gain10/1 -> Scope3/1, Mux4/1  "wm"
  Sum7/1 -> Scope4/1, Mux5/1
  Demux4/1 -> Scope22/1, Scope25/1, [LQR_Ud]
  Constant6/1 -> MATLAB Function1/5(Ls)
  Constant2/1 -> MATLAB Function1/1(P)
  [id] -> Scope23/1, Mux4/2
  Mux4/1 -> Product/2
  From8/1 -> Gain7/1
  MATLAB Function1/1(k) -> Data Type Conversion2/1
  [ref_rpm] -> Scope21/1, Sum7/1
  Demux4/2 -> [LQR_Uq], Scope25/2, Scope22/2
  Data Type Conversion3/1 -> Sum8/1
  Constant4/1 -> MATLAB Function1/3(J)
  [id] -> Sum8/2
  Constant9/1 -> Data Type Conversion4/1
  Discrete-Time Integrator5/1 -> Scope/1, Product1/2
  Constant7/1 -> MATLAB Function1/6(B)
  [real_rpm] -> Gain10/1
  [iq] -> Scope23/2, Mux4/3
  Constant8/1 -> Data Type Conversion3/1
  Constant3/1 -> MATLAB Function1/2(Flux)
  Product/1 -> Sum6/2, Scope24/1
  Data Type Conversion4/1 -> Mux5/3
  Gain7/1 -> Data Type Conversion1/1
  Sum6/1 -> Demux4/1
  [real_rpm] -> Scope21/2, Sum7/2
  Mux5/1 -> Discrete-Time Integrator5/1
  Sum8/1 -> Scope27/1, Mux5/2
  Ref_RPM/1 -> [ref_rpm]
  Real_RPM/1 -> [real_rpm]
  id/1 -> [id]
  iq/1 -> [iq]
  [LQR_Ud] -> Ud/1
  [LQR_Uq] -> Uq/1
  Data Type Conversion1/1 -> MATLAB Function1/7(we)
  Constant/1 -> Mux/1
  Constant1/1 -> Mux/2
  Constant10/1 -> Mux/3
  Reshape/1 -> Data Type Conversion5/1
  Mux/1 -> Reshape/1
  Constant11/1 -> Mux/4
  Constant12/1 -> Mux/5
  Constant13/1 -> Mux/6
  Data Type Conversion5/1 -> Scope2/1, Product1/1, Scope26/1, Product/1
  Product1/1 -> Scope1/1, Sum6/1

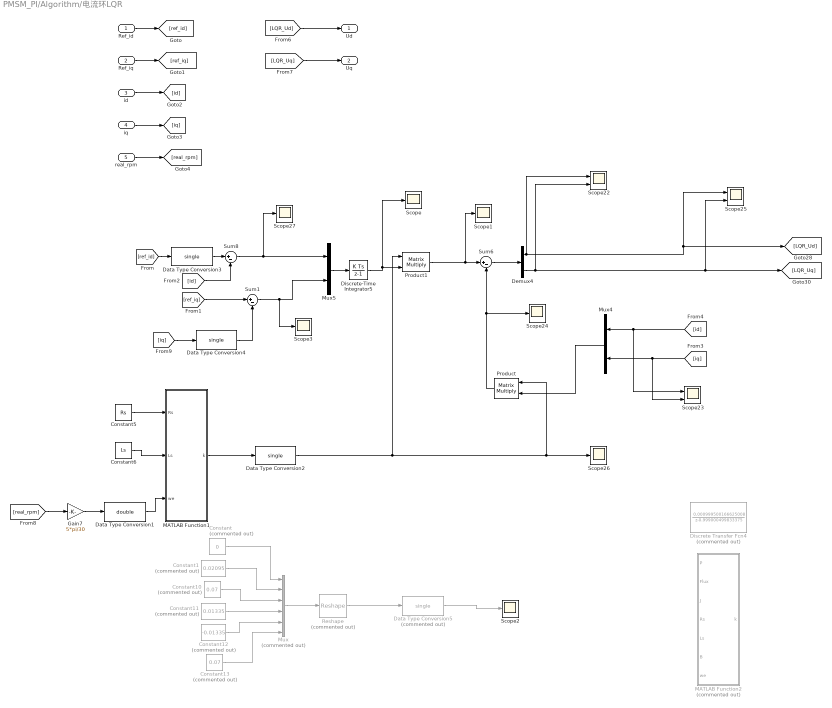
== system PMSM_PI/Algorithm/电流环LQR ==
  Ref_id : Inport
  Ref_iq : Inport  Port=2
  id : Inport  Port=3
  iq : Inport  Port=4
  real_rpm : Inport  Port=5
  Constant : Constant  Commented=on  Value=0  SampleTime=Ts
  Constant1 : Constant  Commented=on  Value=0.02095  SampleTime=Ts
  Constant10 : Constant  Commented=on  Value=0.07  SampleTime=Ts
  Constant11 : Constant  Commented=on  Value=0.01335  SampleTime=Ts
  Constant12 : Constant  Commented=on  Value=-0.01335  SampleTime=Ts
  Constant13 : Constant  Commented=on  Value=0.07  SampleTime=Ts
  Constant5 : Constant  Value=Rs  SampleTime=Ts
  Constant6 : Constant  Value=Ls  SampleTime=Ts
  Data Type Conversion1 : DataTypeConversion  OutDataTypeStr=double  SaturateOnIntegerOverflow=off  RndMeth=Floor
  Data Type Conversion2 : DataTypeConversion  OutDataTypeStr=single  SaturateOnIntegerOverflow=off  RndMeth=Floor
  Data Type Conversion3 : DataTypeConversion  OutDataTypeStr=single  SaturateOnIntegerOverflow=off  RndMeth=Floor
  Data Type Conversion4 : DataTypeConversion  OutDataTypeStr=single  SaturateOnIntegerOverflow=off  RndMeth=Floor
  Data Type Conversion5 : DataTypeConversion  Commented=on  OutDataTypeStr=single  SaturateOnIntegerOverflow=off  RndMeth=Floor
  Demux4 : Demux  Outputs=2
  Discrete Transfer Fcn4 : DiscreteTransferFcn  Commented=on  Numerator=[0.000999500166625008]  Denominator=[1 -0.999000499833375]
  Discrete-Time Integrator5 : DiscreteIntegrator  gainval=50  SampleTime=-1  ICPrevOutput=DiscIntNeverNeededParam  ICPrevScaledInput=DiscIntNeverNeededParam
  Gain7 : Gain  Gain=5*pi/30
  MATLAB Function1 : MATLAB Function  TreatAsAtomicUnit=on
  MATLAB Function2 : MATLAB Function  Commented=on  TreatAsAtomicUnit=on
  Mux : Mux  Commented=on  Inputs=6
  Mux4 : Mux  Inputs=2
  Mux5 : Mux  Inputs=2
  Product : Product  Multiplication=Matrix(*)
  Product1 : Product  Multiplication=Matrix(*)
  Reshape : Reshape  Commented=on  OutputDimensionality=Customize  OutputDimensions=[2,3]
  Scope{,1..3,24,26..27} (7 alike) : Scope
  Scope22 : Scope  NumInputPorts=2
  Scope23 : Scope  NumInputPorts=2
  Scope25 : Scope  NumInputPorts=2
  Sum1 : Sum  Inputs=|+-
  Sum6 : Sum  Inputs=|+-
  Sum8 : Sum  Inputs=|+-
  Ud : Outport
  Uq : Outport  Port=2
  wires:
  Product1/1 -> Sum6/1, Scope1/1
  Data Type Conversion5/1 -> Scope2/1
  Constant13/1 -> Mux/6
  Constant12/1 -> Mux/5
  Constant11/1 -> Mux/4
  Mux/1 -> Reshape/1
  Reshape/1 -> Data Type Conversion5/1
  Constant10/1 -> Mux/3
  Constant1/1 -> Mux/2
  Constant/1 -> Mux/1
  Data Type Conversion1/1 -> MATLAB Function1/3(we)
  [LQR_Uq] -> Uq/1
  [LQR_Ud] -> Ud/1
  iq/1 -> [iq]
  id/1 -> [id]
  Ref_iq/1 -> [ref_iq]
  Ref_id/1 -> [ref_id]
  Sum8/1 -> Scope27/1, Mux5/1
  Mux5/1 -> Discrete-Time Integrator5/1
  Sum6/1 -> Demux4/1
  Gain7/1 -> Data Type Conversion1/1
  Data Type Conversion4/1 -> Sum1/2
  Product/1 -> Scope24/1, Sum6/2
  [ref_id] -> Data Type Conversion3/1
  [iq] -> Mux4/2, Scope23/2
  Discrete-Time Integrator5/1 -> Product1/2, Scope/1
  [iq] -> Data Type Conversion4/1
  [id] -> Sum8/2
  Data Type Conversion3/1 -> Sum8/1
  Demux4/2 -> Scope22/2, Scope25/2, [LQR_Uq]
  MATLAB Function1/1(k) -> Data Type Conversion2/1
  [real_rpm] -> Gain7/1
  Mux4/1 -> Product/2
  [id] -> Mux4/1, Scope23/1
  Constant6/1 -> MATLAB Function1/2(Ls)
  Demux4/1 -> [LQR_Ud], Scope25/1, Scope22/1
  Constant5/1 -> MATLAB Function1/1(Rs)
  Data Type Conversion2/1 -> Product1/1, Product/1, Scope26/1
  [ref_iq] -> Sum1/1
  Sum1/1 -> Scope3/1, Mux5/2
  real_rpm/1 -> [real_rpm]

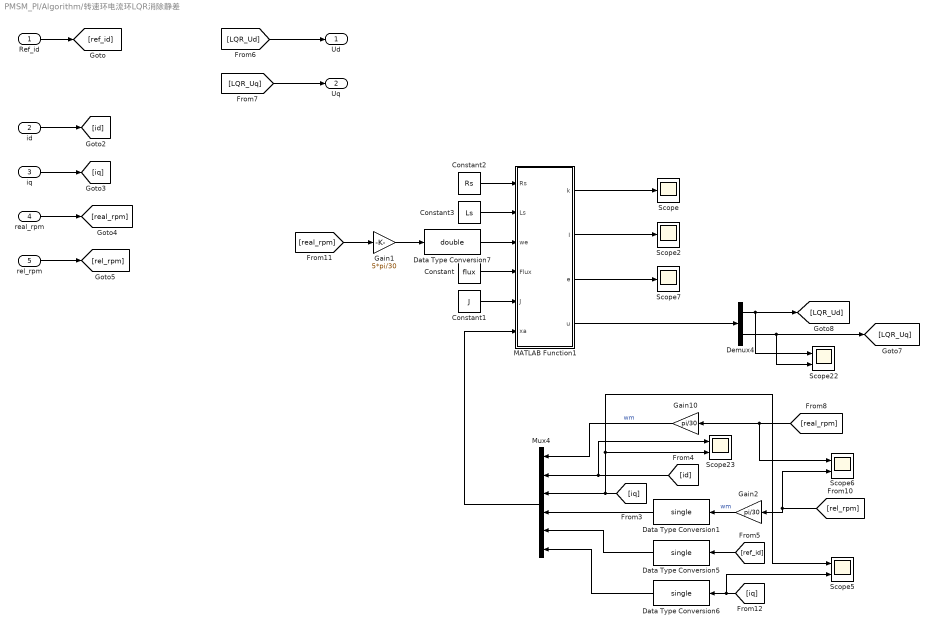
== system PMSM_PI/Algorithm/转速环电流环LQR消除静差 ==
  Ref_id : Inport
  id : Inport  Port=2
  iq : Inport  Port=3
  real_rpm : Inport  Port=4
  rel_rpm : Inport  Port=5
  Constant : Constant  Value=flux  SampleTime=Ts
  Constant1 : Constant  Value=J  SampleTime=Ts
  Constant2 : Constant  Value=Rs  SampleTime=Ts
  Constant3 : Constant  Value=Ls  SampleTime=Ts
  Data Type Conversion1 : DataTypeConversion  OutDataTypeStr=single  SaturateOnIntegerOverflow=off  RndMeth=Floor
  Data Type Conversion5 : DataTypeConversion  OutDataTypeStr=single  SaturateOnIntegerOverflow=off  RndMeth=Floor
  Data Type Conversion6 : DataTypeConversion  OutDataTypeStr=single  SaturateOnIntegerOverflow=off  RndMeth=Floor
  Data Type Conversion7 : DataTypeConversion  OutDataTypeStr=double  SaturateOnIntegerOverflow=off  RndMeth=Floor
  Demux4 : Demux  Outputs=2
  Gain1 : Gain  Gain=5*pi/30
  Gain10 : Gain  Gain=pi/30
  Gain2 : Gain  Gain=pi/30
  MATLAB Function1 : MATLAB Function  TreatAsAtomicUnit=on
  Mux4 : Mux  Inputs=6
  Scope : Scope
  Scope2 : Scope
  Scope{5..6,22..23} (4 alike) : Scope  NumInputPorts=2
  Scope7 : Scope
  Ud : Outport
  Uq : Outport  Port=2
  wires:
  MATLAB Function1/3(e) -> Scope7/1
  Gain2/1 -> Data Type Conversion1/1  "wm"
  Constant1/1 -> MATLAB Function1/5(J)
  Data Type Conversion1/1 -> Mux4/4
  [rel_rpm] -> Gain2/1, Scope6/2
  rel_rpm/1 -> [rel_rpm]
  [real_rpm] -> Gain10/1, Scope6/1
  Gain10/1 -> Mux4/1  "wm"
  real_rpm/1 -> [real_rpm]
  Demux4/1 -> [LQR_Ud], Scope22/1
  [id] -> Scope23/1, Mux4/2
  Mux4/1 -> MATLAB Function1/6(xa)
  MATLAB Function1/1(k) -> Scope/1
  Demux4/2 -> [LQR_Uq], Scope22/2
  [iq] -> Mux4/3, Scope23/2, Scope5/1
  Ref_id/1 -> [ref_id]
  id/1 -> [id]
  iq/1 -> [iq]
  [LQR_Ud] -> Ud/1
  [LQR_Uq] -> Uq/1
  [ref_id] -> Data Type Conversion5/1
  Data Type Conversion5/1 -> Mux4/5
  Data Type Conversion6/1 -> Mux4/6
  [iq] -> Data Type Conversion6/1, Scope5/2
  MATLAB Function1/2(I) -> Scope2/1
  Data Type Conversion7/1 -> MATLAB Function1/3(we)
  Gain1/1 -> Data Type Conversion7/1
  [real_rpm] -> Gain1/1
  Constant3/1 -> MATLAB Function1/2(Ls)
  Constant2/1 -> MATLAB Function1/1(Rs)
  Constant/1 -> MATLAB Function1/4(Flux)
  MATLAB Function1/4(u) -> Demux4/1

== system PMSM_PI/Algorithm/Algorithm/Clark_Trans ==
  note: $u_\alpha=\frac{2}{3}(u_a-\frac{1}{2}u_b-\frac{1}{2}u_c ) \\ u_\beta=\frac{2}{3}(\frac{\sqrt{3}}{2}u_b-\frac{\sqrt{3}}{2}u_c)$
  note: Clark_Transform
  Ia : Inport  OutDataTypeStr=single
  Ib : Inport  Port=2  OutDataTypeStr=single
  Ic : Inport  Port=3  OutDataTypeStr=single
  Add : Sum  Inputs=+-  OutDataTypeStr=single
  Add1 : Sum  OutDataTypeStr=single
  Add2 : Sum  Inputs=+-  OutDataTypeStr=single
  Gain : Gain  Gain=0.5  OutDataTypeStr=single
  Gain1 : Gain  Gain=sqrt(3)/2  OutDataTypeStr=single
  Gain2 : Gain  Gain=2/3  OutDataTypeStr=single
  Gain3 : Gain  Gain=2/3  OutDataTypeStr=single
  I_alpha : Outport  OutDataTypeStr=single
  I_beta : Outport  Port=2  OutDataTypeStr=single
  wires:
  Ia/1 -> Add/1
  Gain/1 -> Add/2
  Ib/1 -> Add1/1, Add2/1
  Ic/1 -> Add1/2, Add2/2
  Add2/1 -> Gain1/1
  Add1/1 -> Gain/1
  Add/1 -> Gain2/1
  Gain2/1 -> I_alpha/1
  Gain1/1 -> Gain3/1
  Gain3/1 -> I_beta/1
